simulink model "smd.slx"  (R2026a)
settings: Solver=VariableStepAuto

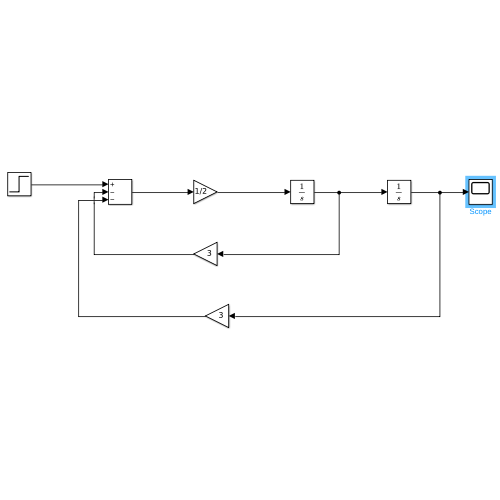
[thumbnail: Simulink's stored preview of the top-level diagram]
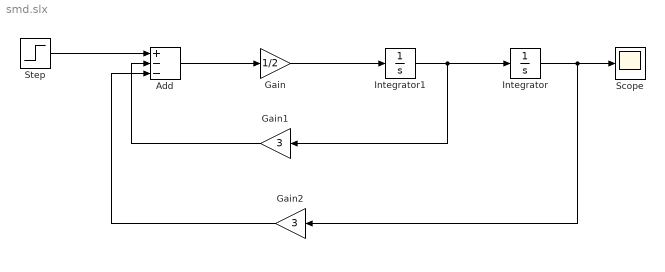
== system smd.slx ==
  Add : Sum  Inputs=+--
  Gain : Gain  Gain=1/2
  Gain1 : Gain  Gain=3
  Gain2 : Gain  Gain=3
  Integrator : Integrator
  Integrator1 : Integrator
  Scope : Scope
      settings: ActiveDisplayYMinimum=-1.0584803183234097  ActiveDisplayYMaximum=2.4048195356737825
  Step : Step  SampleTime=0
  wires:
  Step/1 -> Add/1
  Add/1 -> Gain/1
  Gain/1 -> Integrator1/1
  Integrator1/1 -> Gain1/1, Integrator/1
  Integrator/1 -> Gain2/1, Scope/1
  Gain1/1 -> Add/2
  Gain2/1 -> Add/3
